simulink model "acc_model"  (R2024b)
settings: Solver=ode4  StartTime=0.0  StopTime=40  FixedStep=0.01  RelTol=1e-3
libraries: simulink x1
settings Model: Creator=User  LastModifiedBy=User

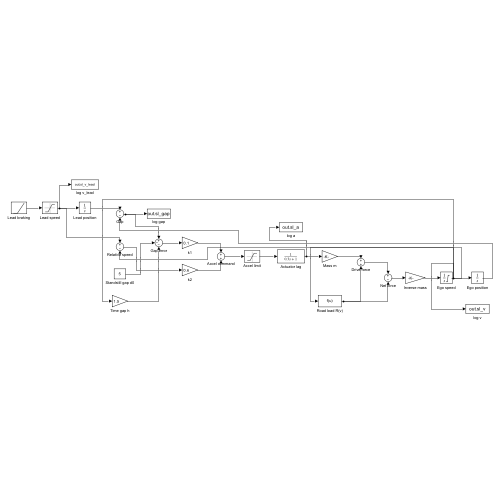
[thumbnail: Simulink's stored preview of the top-level diagram]
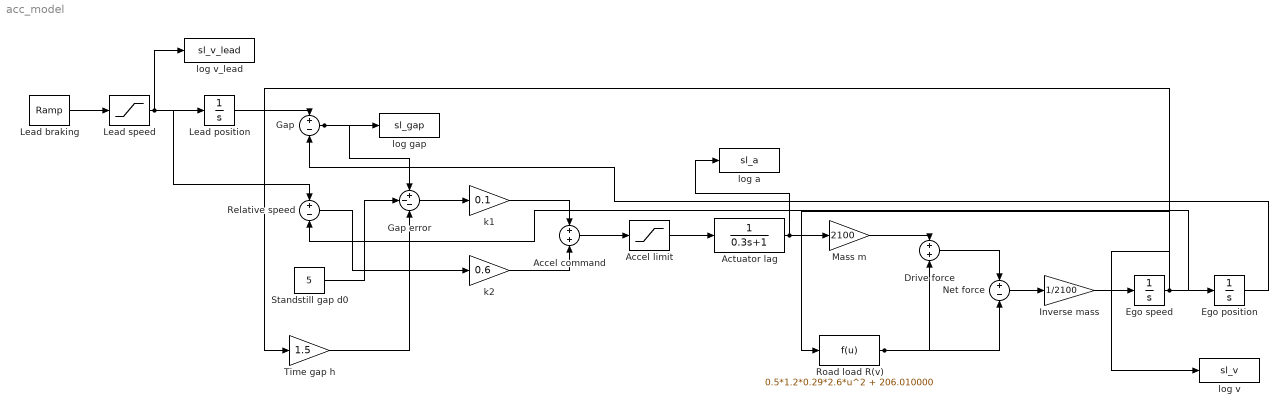
== system acc_model ==
  Accel command : Sum
  Accel limit : Saturate  UpperLimit=2  LowerLimit=-3.5
  Actuator lag : TransferFcn  Numerator=1  Denominator=[0.3 1]
  Drive force : Sum
  Ego position : Integrator
  Ego speed : Integrator  InitialCondition=27.77777778  LimitOutput=on  LowerSaturationLimit=0
  Gap : Sum  Inputs=+-
  Gap error : Sum  Inputs=+--
  Inverse mass : Gain  Gain=1/2100
  Lead braking : simulink/Sources/Ramp  slope=-3  start=5  InitialOutput=27.77777778
  Lead position : Integrator  InitialCondition=46.66666667
  Lead speed : Saturate  UpperLimit=27.77777778  LowerLimit=16.66666667
  Mass m : Gain  Gain=2100
  Net force : Sum  Inputs=+-
  Relative speed : Sum  Inputs=+-
  Road load R(v) : Fcn  Expr=0.5*1.2*0.29*2.6*u^2 + 206.010000
  Standstill gap d0 : Constant  Value=5
  Time gap h : Gain  Gain=1.5
  k1 : Gain  Gain=0.1
  k2 : Gain  Gain=0.6
  log a : ToWorkspace  VariableName=sl_a  SampleTime=-1
  log gap : ToWorkspace  VariableName=sl_gap  SampleTime=-1
  log v : ToWorkspace  VariableName=sl_v  SampleTime=-1
  log v_lead : ToWorkspace  VariableName=sl_v_lead  SampleTime=-1
  wires:
  Lead braking/1 -> Lead speed/1
  Lead speed/1 -> Lead position/1, Relative speed/1, log v_lead/1
  Lead position/1 -> Gap/1
  Ego position/1 -> Gap/2
  Ego speed/1 -> Relative speed/2, Time gap h/1, Road load R(v)/1, Ego position/1, log v/1
  Gap/1 -> Gap error/1, log gap/1
  Standstill gap d0/1 -> Gap error/2
  Time gap h/1 -> Gap error/3
  Gap error/1 -> k1/1
  Relative speed/1 -> k2/1
  k1/1 -> Accel command/1
  k2/1 -> Accel command/2
  Accel command/1 -> Accel limit/1
  Accel limit/1 -> Actuator lag/1
  Actuator lag/1 -> Mass m/1, log a/1
  Mass m/1 -> Drive force/1
  Road load R(v)/1 -> Drive force/2, Net force/2
  Drive force/1 -> Net force/1
  Net force/1 -> Inverse mass/1
  Inverse mass/1 -> Ego speed/1
